simulink model "MSFP2NFGA"  (R2026b)
settings: Solver=ode15s  MaxStep=1E-2
libraries: slpidlib x2
settings Model: LastModifiedBy=Neltzon Farid
settings DataIOCC: DSMLogging=off  ReturnWorkspaceOutputs=off  SaveOutput=off  SignalLogging=off  TimeSaveName=t
settings DebuggingCC: AlgebraicLoopMsg=none  ArtificialAlgebraicLoopMsg=none  MaxConsecutiveZCsMsg=none

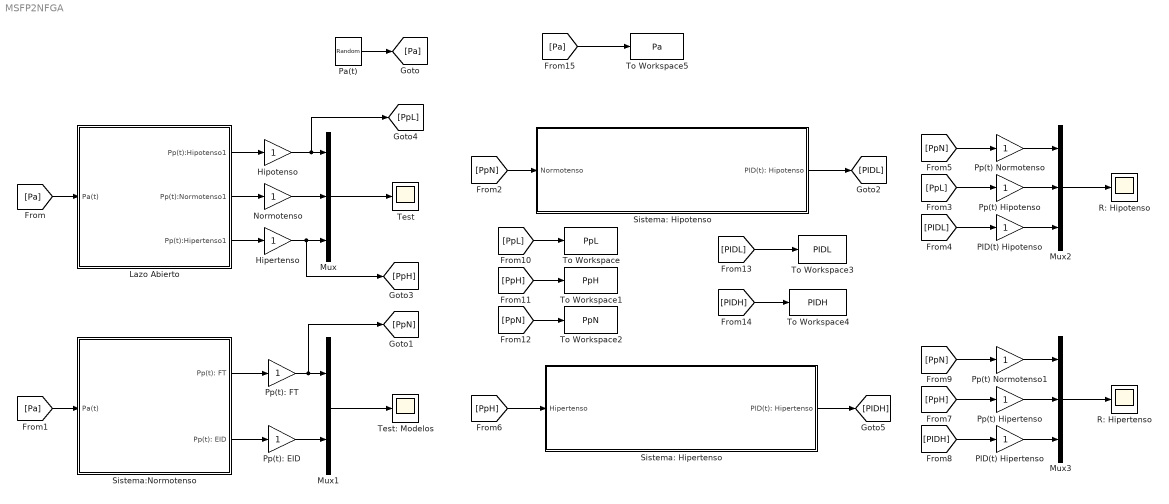
== system MSFP2NFGA ==
  Hipertenso : Gain
  Hipotenso : Gain
  Lazo Abierto : Subsystem
  Mux : Mux  Inputs=3
  Mux1 : Mux  Inputs=2
  Mux2 : Mux  Inputs=3
  Mux3 : Mux  Inputs=3
  Normotenso : Gain
  PID(t) Hipertenso : Gain
  PID(t) Hipotenso : Gain
  Pa(t) : UniformRandomNumber  Minimum=-0.2  Seed=106  SampleTime=0.1
  Pp(t) Hipertenso : Gain
  Pp(t) Hipotenso : Gain
  Pp(t) Normotenso : Gain
  Pp(t) Normotenso1 : Gain
  Pp(t): EID : Gain
  Pp(t): FT : Gain
  R: Hipertenso : Scope
      settings: ActiveDisplayYMinimum=-0.43325479696703184  ActiveDisplayYMaximum=1.128182061765969  YLabel=V(t)  DataLoggingVariableName=ScopeData3
  R: Hipotenso : Scope
      settings: ActiveDisplayYMinimum=-0.43325479696703184  ActiveDisplayYMaximum=1.128182061765969  YLabel=V(t)  DataLoggingVariableName=ScopeData2
  Sistema: Hipertenso : Subsystem
  Sistema: Hipotenso : Subsystem
  Sistema:Normotenso : Subsystem
  Test : Scope
      settings: ActiveDisplayYMinimum=-0.09733221667087022  ActiveDisplayYMaximum=1.1123823568001729  YLabel=V(t)
  Test: Modelos : Scope
      settings: ActiveDisplayYMinimum=-0.74388631619415779  ActiveDisplayYMaximum=1.6755428307479283  YLabel=V(t)
  To Workspace : ToWorkspace  VariableName=PpL  SampleTime=-1
  To Workspace1 : ToWorkspace  VariableName=PpH  SampleTime=-1
  To Workspace2 : ToWorkspace  VariableName=PpN  SampleTime=-1
  To Workspace3 : ToWorkspace  VariableName=PIDL  SampleTime=-1
  To Workspace4 : ToWorkspace  VariableName=PIDH  SampleTime=-1
  To Workspace5 : ToWorkspace  VariableName=Pa  SampleTime=-1
  wires:
  [Pa] -> Lazo Abierto/1(Pa(t))
  Lazo Abierto/1(Pp(t):Hipotenso1) -> Hipotenso/1
  Lazo Abierto/2(Pp(t):Normotenso1) -> Normotenso/1
  Lazo Abierto/3(Pp(t):Hipertenso1) -> Hipertenso/1
  Pa(t)/1 -> [Pa]
  Mux/1 -> Test/1
  Hipotenso/1 -> [PpL], Mux/1
  Normotenso/1 -> Mux/2
  Hipertenso/1 -> [PpH], Mux/3
  Mux1/1 -> Test: Modelos/1
  Sistema:Normotenso/1(Pp(t): FT) -> Pp(t): FT/1
  Sistema:Normotenso/2(Pp(t): EID) -> Pp(t): EID/1
  [Pa] -> Sistema:Normotenso/1(Pa(t))
  [PpN] -> Sistema: Hipotenso/1(Normotenso)
  Sistema: Hipotenso/1(PID(t): Hipotenso) -> [PIDL]
  Mux2/1 -> R: Hipotenso/1
  [PpL] -> Pp(t) Hipotenso/1
  [PpN] -> Pp(t) Normotenso/1
  [PIDL] -> PID(t) Hipotenso/1
  PID(t) Hipotenso/1 -> Mux2/3
  Pp(t) Hipotenso/1 -> Mux2/2
  Pp(t) Normotenso/1 -> Mux2/1
  Pp(t): FT/1 -> [PpN], Mux1/1
  Sistema: Hipertenso/1(PID(t): Hipertenso) -> [PIDH]
  [PpH] -> Sistema: Hipertenso/1(Hipertenso)
  [PpH] -> Pp(t) Hipertenso/1
  Mux3/1 -> R: Hipertenso/1
  Pp(t) Hipertenso/1 -> Mux3/2
  PID(t) Hipertenso/1 -> Mux3/3
  Pp(t) Normotenso1/1 -> Mux3/1
  [PIDH] -> PID(t) Hipertenso/1
  [PpN] -> Pp(t) Normotenso1/1
  [PpH] -> To Workspace1/1
  [PpN] -> To Workspace2/1
  [PpL] -> To Workspace/1
  [PIDL] -> To Workspace3/1
  [PIDH] -> To Workspace4/1
  Pp(t): EID/1 -> Mux1/2
  [Pa] -> To Workspace5/1

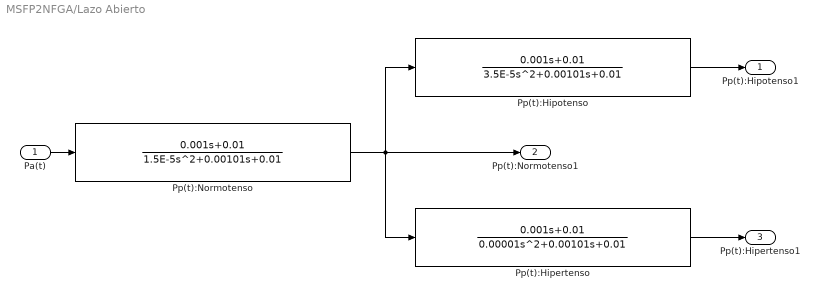
== system MSFP2NFGA/Lazo Abierto ==
  Pa(t) : Inport
  Pp(t):Hipertenso : TransferFcn  Numerator=[0.001,0.01]  Denominator=[0.00001,0.00101,0.01]
  Pp(t):Hipotenso : TransferFcn  Numerator=[0.001,0.01]  Denominator=[3.5E-5,0.00101,0.01]
  Pp(t):Normotenso : TransferFcn  Numerator=[0.001,0.01]  Denominator=[1.5E-5,0.00101,0.01]
  Pp(t):Hipotenso1 : Outport
  Pp(t):Normotenso1 : Outport  Port=2
  Pp(t):Hipertenso1 : Outport  Port=3
  wires:
  Pp(t):Normotenso/1 -> Pp(t):Hipertenso/1, Pp(t):Hipotenso/1, Pp(t):Normotenso1/1
  Pa(t)/1 -> Pp(t):Normotenso/1
  Pp(t):Hipertenso/1 -> Pp(t):Hipertenso1/1
  Pp(t):Hipotenso/1 -> Pp(t):Hipotenso1/1

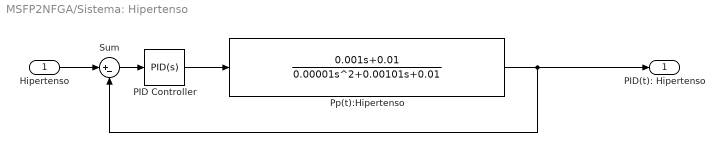
== system MSFP2NFGA/Sistema: Hipertenso ==
  Hipertenso : Inport
  PID Controller : slpidlib/PID Controller  Controller=PID  Form=Parallel  TimeDomain=Continuous-time  UseExternalTs=off  SampleTime=-1  IntegratorMethod=Forward Euler  FilterMethod=Forward Euler  ControllerParametersSource=internal  P=129.978567122813  I=312762.858715908  UseKiTs=off  D=0.00174611348908487  UseExternalDerivativeSource=off  N=49610.1326532739  UseFilter=on  TunerSelectOption=Transfer Function Based (PID Tuner App)  InitialConditionSource=internal  InitialConditionForIntegrator=0  InitialConditionForFilter=0  DifferentiatorICPrevScaledInput=0  ExternalReset=none  TrackingMode=off  Kt=1  LimitOutput=off  SatLimitsSource=internal  UpperSaturationLimit=inf  LowerSaturationLimit=-inf  LinearizeAsGain=on  AntiWindupMode=none  Kb=1  LimitIntegrator=off  UpperIntegratorSaturationLimit=inf  LowerIntegratorSaturationLimit=-inf  POutMin=[]  POutMax=[]  IOutMin=[]  IOutMax=[]  DOutMin=[]  DOutMax=[]  NOutMin=[]  NOutMax=[]  SumOutMin=[]  SumOutMax=[]  SaturationOutMin=[]  SaturationOutMax=[]  PParamMin=[]  PParamMax=[]  IParamMin=[]  IParamMax=[]  DParamMin=[]  DParamMax=[]  NParamMin=[]  NParamMax=[]  KbParamMin=[]  KbParamMax=[]  KtParamMin=[]  KtParamMax=[]  KbOutMin=[]  KbOutMax=[]  KtOutMin=[]  KtOutMax=[]  IntegratorOutMin=[]  IntegratorOutMax=[]  FilterOutMin=[]  FilterOutMax=[]  SumI1OutMin=[]  SumI1OutMax=[]  SumI2OutMin=[]  SumI2OutMax=[]  SumI3OutMin=[]  SumI3OutMax=[]  SumI4OutMin=[]  SumI4OutMax=[]  SumDOutMin=[]  SumDOutMax=[]  DifferentiatorOutMin=[]  DifferentiatorOutMax=[]  FilterDiffOutCoefMin=[]  FilterDiffOutCoefMax=[]  ReciprocalOutMin=[]  ReciprocalOutMax=[]  SumDenOutMin=[]  SumDenOutMax=[]  SumNumOutMin=[]  SumNumOutMax=[]  DivideOutMin=[]  DivideOutMax=[]  UdiffTsProdOutMin=[]  UdiffTsProdOutMax=[]  NTsProdOutMin=[]  NTsProdOutMax=[]  UintegralTsProdOutMin=[]  UintegralTsProdOutMax=[]  UngainTsProdOutMin=[]  UngainTsProdOutMax=[]  ClampingZeroOutDataTypeStr=Inherit: Inherit via back propagation  ClampingZeroOutMin=[]  ClampingZeroOutMax=[]  FilterDenConstantOutDataTypeStr=Inherit: Inherit via back propagation  FilterDenConstantOutMin=[]  FilterDenConstantOutMax=[]  PCopyOutDataTypeStr=Inherit: Inherit via back propagation  PCopyOutMin=[]  PCopyOutMax=[]  NCopyOutDataTypeStr=Inherit: Inherit via back propagation  NCopyOutMin=[]  NCopyOutMax=[]  IntegratorContinuousStateAttributes=''  IntegratorStateMustResolveToSignalObject=off  IntegratorRTWStateStorageClass=Auto  FilterContinuousStateAttributes=''  FilterStateMustResolveToSignalObject=off  FilterRTWStateStorageClass=Auto  ParallelPVariant=InternalParameters  IdealPVariant=Disabled  IVariant=InternalParameters  DVariant=InternalParameters  IntegratorVariant=Continuous  SatVariant=Disabled  AWVariant=Passthrough  PCopyVariant=Disabled  TRVariant=Disabled  FdbkBlocksVariant=Forward  IdealPFdbkVariant=Disabled  SatFdbkVariant=Disabled  DerivativeFilterVariant=ContFilter  NVariant=InternalParameters  NCopyVariant=Disabled  FilterICVariant=InternalICsFilter  IntegratorICVariant=InternalICs  ExternalResetVariant=Disabled  TRSumVariant=Passthrough  SumFdbkVariant=Disabled  SumVariant=Sum_PID  TsampFilterVariant=InternalTs  TsampNgainVariant=Passthrough  TsampIntegralVariant=Disabled_SignalSpec  ExternalSaturationOutDataTypeStr=Inherit: Same as second input  DerivativeSourceVariant=ErrorSignal  PreIntVariant=InternalPreInt
  Pp(t):Hipertenso : TransferFcn  Numerator=[0.001,0.01]  Denominator=[0.00001,0.00101,0.01]
  Sum : Sum  Inputs=|+-
  PID(t): Hipertenso : Outport
  wires:
  Sum/1 -> PID Controller/1
  PID Controller/1 -> Pp(t):Hipertenso/1
  Hipertenso/1 -> Sum/1
  Pp(t):Hipertenso/1 -> Sum/2, PID(t): Hipertenso/1

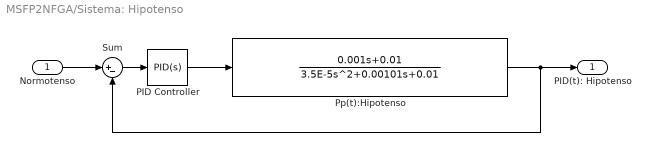
== system MSFP2NFGA/Sistema: Hipotenso ==
  Normotenso : Inport
  PID Controller : slpidlib/PID Controller  Controller=PID  Form=Parallel  TimeDomain=Continuous-time  UseExternalTs=off  SampleTime=-1  IntegratorMethod=Forward Euler  FilterMethod=Forward Euler  ControllerParametersSource=internal  P=459.759940880943  I=1118300.3780121  UseKiTs=off  D=0.00626733381384696  UseExternalDerivativeSource=off  N=50197.1654063455  UseFilter=on  TunerSelectOption=Transfer Function Based (PID Tuner App)  InitialConditionSource=internal  InitialConditionForIntegrator=0  InitialConditionForFilter=0  DifferentiatorICPrevScaledInput=0  ExternalReset=none  TrackingMode=off  Kt=1  LimitOutput=off  SatLimitsSource=internal  UpperSaturationLimit=inf  LowerSaturationLimit=-inf  LinearizeAsGain=on  AntiWindupMode=none  Kb=1  LimitIntegrator=off  UpperIntegratorSaturationLimit=inf  LowerIntegratorSaturationLimit=-inf  POutMin=[]  POutMax=[]  IOutMin=[]  IOutMax=[]  DOutMin=[]  DOutMax=[]  NOutMin=[]  NOutMax=[]  SumOutMin=[]  SumOutMax=[]  SaturationOutMin=[]  SaturationOutMax=[]  PParamMin=[]  PParamMax=[]  IParamMin=[]  IParamMax=[]  DParamMin=[]  DParamMax=[]  NParamMin=[]  NParamMax=[]  KbParamMin=[]  KbParamMax=[]  KtParamMin=[]  KtParamMax=[]  KbOutMin=[]  KbOutMax=[]  KtOutMin=[]  KtOutMax=[]  IntegratorOutMin=[]  IntegratorOutMax=[]  FilterOutMin=[]  FilterOutMax=[]  SumI1OutMin=[]  SumI1OutMax=[]  SumI2OutMin=[]  SumI2OutMax=[]  SumI3OutMin=[]  SumI3OutMax=[]  SumI4OutMin=[]  SumI4OutMax=[]  SumDOutMin=[]  SumDOutMax=[]  DifferentiatorOutMin=[]  DifferentiatorOutMax=[]  FilterDiffOutCoefMin=[]  FilterDiffOutCoefMax=[]  ReciprocalOutMin=[]  ReciprocalOutMax=[]  SumDenOutMin=[]  SumDenOutMax=[]  SumNumOutMin=[]  SumNumOutMax=[]  DivideOutMin=[]  DivideOutMax=[]  UdiffTsProdOutMin=[]  UdiffTsProdOutMax=[]  NTsProdOutMin=[]  NTsProdOutMax=[]  UintegralTsProdOutMin=[]  UintegralTsProdOutMax=[]  UngainTsProdOutMin=[]  UngainTsProdOutMax=[]  ClampingZeroOutDataTypeStr=Inherit: Inherit via back propagation  ClampingZeroOutMin=[]  ClampingZeroOutMax=[]  FilterDenConstantOutDataTypeStr=Inherit: Inherit via back propagation  FilterDenConstantOutMin=[]  FilterDenConstantOutMax=[]  PCopyOutDataTypeStr=Inherit: Inherit via back propagation  PCopyOutMin=[]  PCopyOutMax=[]  NCopyOutDataTypeStr=Inherit: Inherit via back propagation  NCopyOutMin=[]  NCopyOutMax=[]  IntegratorContinuousStateAttributes=''  IntegratorStateMustResolveToSignalObject=off  IntegratorRTWStateStorageClass=Auto  FilterContinuousStateAttributes=''  FilterStateMustResolveToSignalObject=off  FilterRTWStateStorageClass=Auto  ParallelPVariant=InternalParameters  IdealPVariant=Disabled  IVariant=InternalParameters  DVariant=InternalParameters  IntegratorVariant=Continuous  SatVariant=Disabled  AWVariant=Passthrough  PCopyVariant=Disabled  TRVariant=Disabled  FdbkBlocksVariant=Forward  IdealPFdbkVariant=Disabled  SatFdbkVariant=Disabled  DerivativeFilterVariant=ContFilter  NVariant=InternalParameters  NCopyVariant=Disabled  FilterICVariant=InternalICsFilter  IntegratorICVariant=InternalICs  ExternalResetVariant=Disabled  TRSumVariant=Passthrough  SumFdbkVariant=Disabled  SumVariant=Sum_PID  TsampFilterVariant=InternalTs  TsampNgainVariant=Passthrough  TsampIntegralVariant=Disabled_SignalSpec  ExternalSaturationOutDataTypeStr=Inherit: Same as second input  DerivativeSourceVariant=ErrorSignal  PreIntVariant=InternalPreInt
  Pp(t):Hipotenso : TransferFcn  Numerator=[0.001,0.01]  Denominator=[3.5E-5,0.00101,0.01]
  Sum : Sum  Inputs=|+-
  PID(t): Hipotenso : Outport
  wires:
  Sum/1 -> PID Controller/1
  PID Controller/1 -> Pp(t):Hipotenso/1
  Normotenso/1 -> Sum/1
  Pp(t):Hipotenso/1 -> Sum/2, PID(t): Hipotenso/1

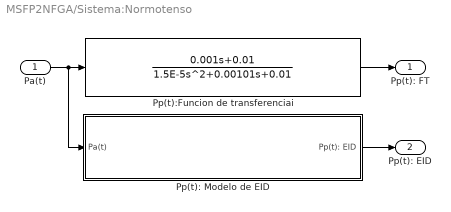
== system MSFP2NFGA/Sistema:Normotenso ==
  Pa(t) : Inport
  Pp(t): Modelo de EID : Subsystem  TreatAsAtomicUnit=on
  Pp(t):Funcion de transferenciai : TransferFcn  Numerator=[0.001,0.01]  Denominator=[1.5E-5,0.00101,0.01]
  Pp(t): FT : Outport
  Pp(t): EID : Outport  Port=2
  wires:
  Pa(t)/1 -> Pp(t): Modelo de EID/1(Pa(t)), Pp(t):Funcion de transferenciai/1
  Pp(t):Funcion de transferenciai/1 -> Pp(t): FT/1
  Pp(t): Modelo de EID/1(Pp(t): EID) -> Pp(t): EID/1

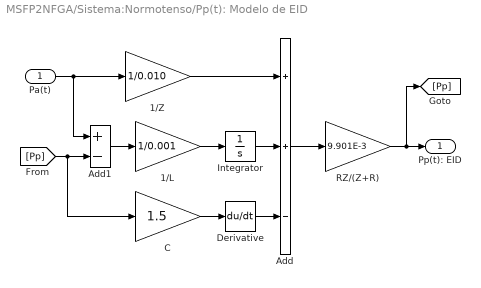
== system MSFP2NFGA/Sistema:Normotenso/Pp(t): Modelo de EID ==
  Pa(t) : Inport
  1/L : Gain  Gain=1/0.001
  1/Z : Gain  Gain=1/0.010
  Add : Sum  Inputs=++-
  Add1 : Sum  Inputs=+-
  C : Gain  Gain=1.5
  Derivative : Derivative
  Integrator : Integrator
  RZ/(Z+R) : Gain  Gain=9.901E-3
  Pp(t): EID : Outport
  wires:
  Add/1 -> RZ/(Z+R)/1
  RZ/(Z+R)/1 -> [Pp], Pp(t): EID/1
  1/Z/1 -> Add/1
  Pa(t)/1 -> Add1/1, 1/Z/1
  [Pp] -> Add1/2, C/1
  1/L/1 -> Integrator/1
  Integrator/1 -> Add/2
  Add1/1 -> 1/L/1
  C/1 -> Derivative/1
  Derivative/1 -> Add/3
